simulink model "ZigzagRobot"  (R2025b)
settings: Solver=VariableStepAuto  StartTime=0.0  StopTime=10.0  RelTol=1e-3
values from neighbouring files (symbols this model uses):
  grid_resolution = 100    [ZigZag_robot_simulation.m]
  initial_radius = R0    (= 1)    [ZigZag_robot_simulation.m]
  Kd_w = 0    [ZigZag_robot_simulation.m]
  Ki_w = 50    [ZigZag_robot_simulation.m]
  Kp_w = 10    [ZigZag_robot_simulation.m]
  L_ax = 0.2    [ZigZag_robot_simulation.m]
  linear_speed_cmd = v_ref_const    (= 0.2)    [ZigZag_robot_simulation.m]
  obs_center = [3; 3]    [ZigZag_robot_simulation.m]
  obstacle_radius = 0.25    [ZigZag_robot_simulation.m]
  r_clean = 0.4    [ZigZag_robot_simulation.m]
  R_w = 0.05    [ZigZag_robot_simulation.m]
  rate_gain = k_R    (= 0.05)    [ZigZag_robot_simulation.m]
  room_length = 20    [ZigZag_robot_simulation.m]
  theta0 = (rand()*2*pi) - pi    [ZigZag_robot_simulation.m]
  x0 = (rand()*room_length) - halfL    [ZigZag_robot_simulation.m]
  y0 = (rand()*room_length) - halfL    [ZigZag_robot_simulation.m]
libraries: slpidlib x2
settings Model: Creator=shubh  LastModifiedBy=shubh

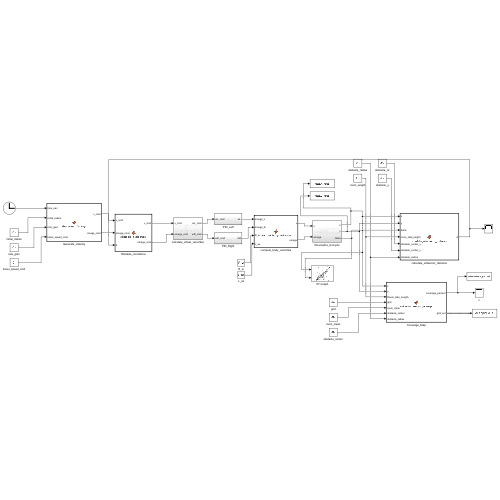
[thumbnail: Simulink's stored preview of the top-level diagram]
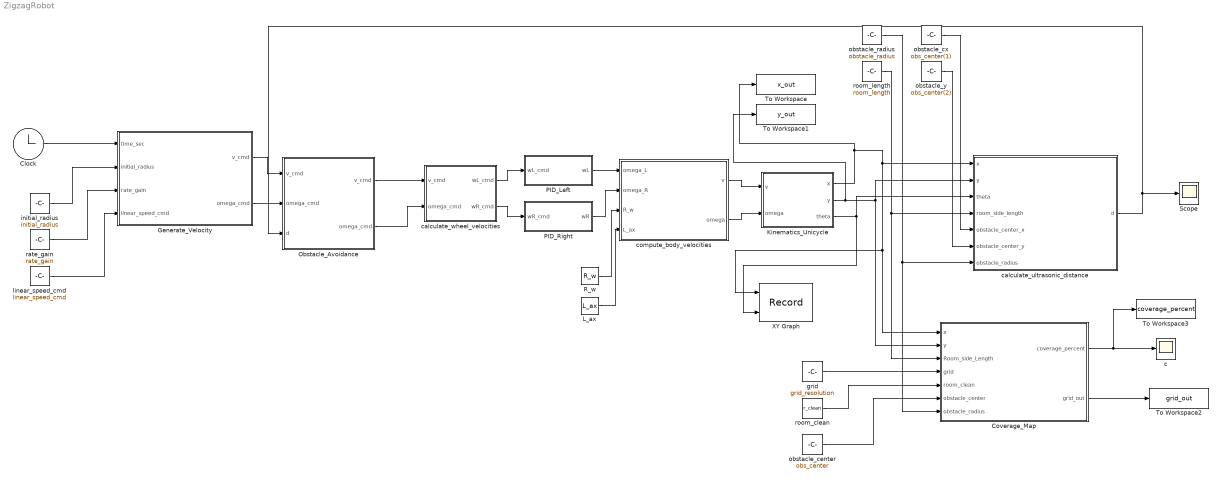
== system ZigzagRobot ==
  Clock : Clock
  Coverage_Map : MATLAB Function  TreatAsAtomicUnit=on
  Generate_Velocity : MATLAB Function  TreatAsAtomicUnit=on
  Kinematics_Unicycle : Subsystem
  L_ax : Constant  Value=L_ax
  Obstacle_Avoidance : MATLAB Function  TreatAsAtomicUnit=on
  PID_Left : Subsystem
  PID_Right : Subsystem
  R_w : Constant  Value=R_w
  Scope : Scope
      settings: ActiveDisplayYMinimum=-1  ActiveDisplayYMaximum=1
  To Workspace : ToWorkspace  VariableName=x_out  SampleTime=-1
  To Workspace1 : ToWorkspace  VariableName=y_out  SampleTime=-1
  To Workspace2 : ToWorkspace  VariableName=grid_out  SaveFormat=Timeseries  SampleTime=-1
  To Workspace3 : ToWorkspace  VariableName=coverage_percent  SaveFormat=Timeseries  SampleTime=-1
  XY Graph : Record  NumPorts=2.0  FileSettingsInternal="{\"entries\":[{\"content\":{\"excelSettings\":{\"content\":{},\"type\":\"Streamout.ExcelSettings\"},\"parquetSettings\":{\"content\":{},\"type\":\"Streamout.ParquetSettings\"}},\"type\":\"Streamout.FileSettingStorage\",\"uuid\":\"\"}],\"packageUris\":[\"http:\\/\\/schema.mathworks.com\\/mf0\\/streamout_blocks\\/R2020a\"],\"version\":\"1.0\"}"  FrameSettings=[0, 0]  Layout=[1 1]  SignalsInternal="{\"entries\":[{\"content\":{\"signals\":[{\"content\":{\"blockPath\":[],\"dimensions\":[1],\"domain\":\"\",\"lineColor\":\"#a2142f\",\"plots\":[ 1 ],\"port\":1,\"signalID\":1,\"signalName\":\"Kinematics_Unicycle:1\"},\"type\":\"RecordBlkView.Signal\",\"uuid\":\"\"},{\"content\":{\"blockPath\":[],\"dimensions\":[1],\"domain\":\"\",\"lineColor\":\"#139fff\",\"plots\":[ 1 ],\"port\":2,\"signalID\":2,\"signalName\":\"Kinematics_Unicycle:3\"},\"type\":\"RecordBlkView.Signal\",\"uuid\":\"\"}]},\"type\":\"RecordBlkView.InputSignals\",\"uuid\":\"\"}],\"packageUris\":[\"http:\\/\\/schema.mathworks.com\\/mf0\\/streamout_blocks\\/R2020a\"],\"version\":\"1.0\"}"  VisualizationBindings="{\"xyplotplugin\":{\"info\":[{\"series\":[{\"bindingParametersList\":[{\"parameter\":\"X-Axis\",\"signalID\":1,\"signalName\":\"Kinematics_Unicycle:1\"},{\"parameter\":\"Y-Axis\",\"signalID\":2,\"signalName\":\"Kinematics_Unicycle:3\"}],\"seriesID\":0}],\"subplotID\":1}]}}"  CompatibilityTag=XY
  c : Scope
      settings: ActiveDisplayYMinimum=-1  ActiveDisplayYMaximum=1
  calculate_ultrasonic_distance : MATLAB Function  TreatAsAtomicUnit=on
  calculate_wheel_velocities : Subsystem
  compute_body_velocities : MATLAB Function  TreatAsAtomicUnit=on
  grid : Constant  Value=grid_resolution
  initial_radius : Constant  Value=initial_radius
  linear_speed_cmd : Constant  Value=linear_speed_cmd
  obstacle_center : Constant  Value=obs_center
  obstacle_cx : Constant  Value=obs_center(1)
  obstacle_radius : Constant  Value=obstacle_radius
  obstacle_y : Constant  Value=obs_center(2)
  rate_gain : Constant  Value=rate_gain
  room_clean : Constant  Value=r_clean
  room_length : Constant  Value=room_length
  wires:
  linear_speed_cmd/1 -> Generate_Velocity/4(linear_speed_cmd)
  calculate_wheel_velocities/1(wL_cmd) -> PID_Left/1(wL_cmd)
  Coverage_Map/2(grid_out) -> To Workspace2/1
  Obstacle_Avoidance/1(v_cmd) -> calculate_wheel_velocities/1(v_cmd)
  room_clean/1 -> Coverage_Map/5(room_clean)
  PID_Right/1(wR) -> compute_body_velocities/2(omega_R)
  Kinematics_Unicycle/2(y) -> To Workspace1/1, calculate_ultrasonic_distance/2(y), Coverage_Map/2(y)
  calculate_ultrasonic_distance/1(d) -> Obstacle_Avoidance/3(d), Scope/1
  room_length/1 -> Coverage_Map/3(Room_side_Length), calculate_ultrasonic_distance/4(room_side_length)
  Obstacle_Avoidance/2(omega_cmd) -> calculate_wheel_velocities/2(omega_cmd)
  L_ax/1 -> compute_body_velocities/4(L_ax)
  obstacle_y/1 -> calculate_ultrasonic_distance/6(obstacle_center_y)
  obstacle_center/1 -> Coverage_Map/6(obstacle_center)
  grid/1 -> Coverage_Map/4(grid)
  Generate_Velocity/1(v_cmd) -> Obstacle_Avoidance/1("v_cmd ")
  obstacle_cx/1 -> calculate_ultrasonic_distance/5(obstacle_center_x)
  calculate_wheel_velocities/2(wR_cmd) -> PID_Right/1(wR_cmd)
  rate_gain/1 -> Generate_Velocity/3(rate_gain)
  Clock/1 -> Generate_Velocity/1(time_sec)
  Kinematics_Unicycle/1(x) -> Coverage_Map/1(x), XY Graph/1, calculate_ultrasonic_distance/1(x), To Workspace/1
  Kinematics_Unicycle/3(theta) -> calculate_ultrasonic_distance/3(theta), XY Graph/2
  PID_Left/1(wL) -> compute_body_velocities/1(omega_L)
  obstacle_radius/1 -> calculate_ultrasonic_distance/7(obstacle_radius), Coverage_Map/7(obstacle_radius)
  Generate_Velocity/2(omega_cmd) -> Obstacle_Avoidance/2("omega_cmd ")
  Coverage_Map/1(coverage_percent) -> To Workspace3/1, c/1
  R_w/1 -> compute_body_velocities/3(R_w)
  compute_body_velocities/2(omega) -> Kinematics_Unicycle/2(omega)
  compute_body_velocities/1(v) -> Kinematics_Unicycle/1(v)
  initial_radius/1 -> Generate_Velocity/2(initial_radius)

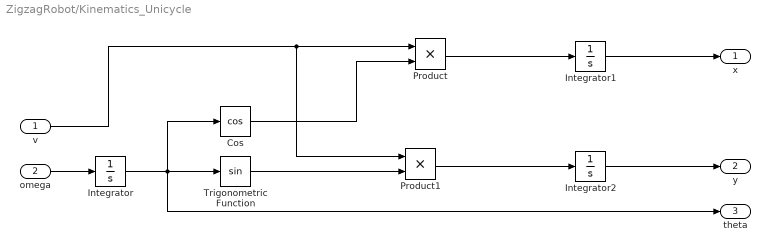
== system ZigzagRobot/Kinematics_Unicycle ==
  v : Inport
  omega : Inport  Port=2
  Cos : Trigonometry  Operator=cos
  Integrator : Integrator  InitialCondition=theta0
  Integrator1 : Integrator  InitialCondition=x0
  Integrator2 : Integrator  InitialCondition=y0
  Product : Product
  Product1 : Product
  Trigonometric Function : Trigonometry
  x : Outport
  y : Outport  Port=2  VectorParamsAs1DForOutWhenUnconnected=off
  theta : Outport  Port=3  VectorParamsAs1DForOutWhenUnconnected=off
  wires:
  omega/1 -> Integrator/1
  Integrator/1 -> theta/1, Trigonometric Function/1, Cos/1
  v/1 -> Product1/1, Product/1
  Cos/1 -> Product/2
  Trigonometric Function/1 -> Product1/2
  Product/1 -> Integrator1/1
  Product1/1 -> Integrator2/1
  Integrator1/1 -> x/1
  Integrator2/1 -> y/1

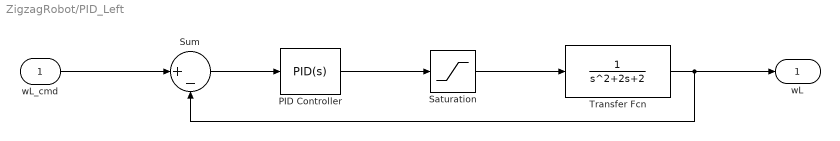
== system ZigzagRobot/PID_Left ==
  wL_cmd : Inport
  PID Controller : slpidlib/PID Controller  Controller=PID  Form=Parallel  TimeDomain=Continuous-time  UseExternalTs=off  SampleTime=-1  IntegratorMethod=Forward Euler  FilterMethod=Forward Euler  ControllerParametersSource=internal  P=Kp_w  I=Ki_w  UseKiTs=off  D=Kd_w  UseExternalDerivativeSource=off  N=100  UseFilter=on  TunerSelectOption=Transfer Function Based (PID Tuner App)  InitialConditionSource=internal  InitialConditionForIntegrator=0  InitialConditionForFilter=0  DifferentiatorICPrevScaledInput=0  ExternalReset=none  TrackingMode=off  Kt=1  LimitOutput=off  SatLimitsSource=internal  UpperSaturationLimit=inf  LowerSaturationLimit=-inf  LinearizeAsGain=on  AntiWindupMode=none  Kb=1  LimitIntegrator=off  UpperIntegratorSaturationLimit=inf  LowerIntegratorSaturationLimit=-inf  POutMin=[]  POutMax=[]  IOutMin=[]  IOutMax=[]  DOutMin=[]  DOutMax=[]  NOutMin=[]  NOutMax=[]  SumOutMin=[]  SumOutMax=[]  SaturationOutMin=[]  SaturationOutMax=[]  PParamMin=[]  PParamMax=[]  IParamMin=[]  IParamMax=[]  DParamMin=[]  DParamMax=[]  NParamMin=[]  NParamMax=[]  KbParamMin=[]  KbParamMax=[]  KtParamMin=[]  KtParamMax=[]  KbOutMin=[]  KbOutMax=[]  KtOutMin=[]  KtOutMax=[]  IntegratorOutMin=[]  IntegratorOutMax=[]  FilterOutMin=[]  FilterOutMax=[]  SumI1OutMin=[]  SumI1OutMax=[]  SumI2OutMin=[]  SumI2OutMax=[]  SumI3OutMin=[]  SumI3OutMax=[]  SumI4OutMin=[]  SumI4OutMax=[]  SumDOutMin=[]  SumDOutMax=[]  DifferentiatorOutMin=[]  DifferentiatorOutMax=[]  FilterDiffOutCoefMin=[]  FilterDiffOutCoefMax=[]  ReciprocalOutMin=[]  ReciprocalOutMax=[]  SumDenOutMin=[]  SumDenOutMax=[]  SumNumOutMin=[]  SumNumOutMax=[]  DivideOutMin=[]  DivideOutMax=[]  UdiffTsProdOutMin=[]  UdiffTsProdOutMax=[]  NTsProdOutMin=[]  NTsProdOutMax=[]  UintegralTsProdOutMin=[]  UintegralTsProdOutMax=[]  UngainTsProdOutMin=[]  UngainTsProdOutMax=[]  ClampingZeroOutDataTypeStr=Inherit: Inherit via back propagation  ClampingZeroOutMin=[]  ClampingZeroOutMax=[]  FilterDenConstantOutDataTypeStr=Inherit: Inherit via back propagation  FilterDenConstantOutMin=[]  FilterDenConstantOutMax=[]  PCopyOutDataTypeStr=Inherit: Inherit via back propagation  PCopyOutMin=[]  PCopyOutMax=[]  NCopyOutDataTypeStr=Inherit: Inherit via back propagation  NCopyOutMin=[]  NCopyOutMax=[]  IntegratorContinuousStateAttributes=''  IntegratorStateMustResolveToSignalObject=off  IntegratorRTWStateStorageClass=Auto  FilterContinuousStateAttributes=''  FilterStateMustResolveToSignalObject=off  FilterRTWStateStorageClass=Auto  ParallelPVariant=InternalParameters  IdealPVariant=Disabled  IVariant=InternalParameters  DVariant=InternalParameters  IntegratorVariant=Continuous  SatVariant=Disabled  AWVariant=Passthrough  PCopyVariant=Disabled  TRVariant=Disabled  FdbkBlocksVariant=Forward  IdealPFdbkVariant=Disabled  SatFdbkVariant=Disabled  DerivativeFilterVariant=ContFilter  NVariant=InternalParameters  NCopyVariant=Disabled  FilterICVariant=InternalICsFilter  IntegratorICVariant=InternalICs  ExternalResetVariant=Disabled  TRSumVariant=Passthrough  SumFdbkVariant=Disabled  SumVariant=Sum_PID  TsampFilterVariant=InternalTs  TsampNgainVariant=Passthrough  TsampIntegralVariant=Disabled_SignalSpec  ExternalSaturationOutDataTypeStr=Inherit: Same as second input  DerivativeSourceVariant=ErrorSignal  PreIntVariant=InternalPreInt
  Saturation : Saturate  UpperLimit=12  LowerLimit=-12
  Sum : Sum  Inputs=|+-
  Transfer Fcn : TransferFcn  Denominator=[1 2 2]
  wL : Outport
  wires:
  Transfer Fcn/1 -> Sum/2, wL/1
  wL_cmd/1 -> Sum/1
  Sum/1 -> PID Controller/1
  PID Controller/1 -> Saturation/1
  Saturation/1 -> Transfer Fcn/1

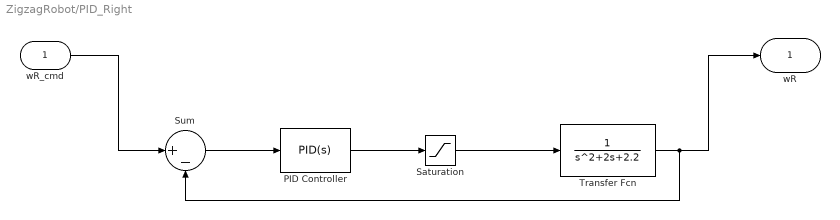
== system ZigzagRobot/PID_Right ==
  wR_cmd : Inport
  PID Controller : slpidlib/PID Controller  Controller=PID  Form=Parallel  TimeDomain=Continuous-time  UseExternalTs=off  SampleTime=-1  IntegratorMethod=Forward Euler  FilterMethod=Forward Euler  ControllerParametersSource=internal  P=Kp_w  I=Ki_w  UseKiTs=off  D=Kd_w  UseExternalDerivativeSource=off  N=100  UseFilter=on  TunerSelectOption=Transfer Function Based (PID Tuner App)  InitialConditionSource=internal  InitialConditionForIntegrator=0  InitialConditionForFilter=0  DifferentiatorICPrevScaledInput=0  ExternalReset=none  TrackingMode=off  Kt=1  LimitOutput=off  SatLimitsSource=internal  UpperSaturationLimit=inf  LowerSaturationLimit=-inf  LinearizeAsGain=on  AntiWindupMode=none  Kb=1  LimitIntegrator=off  UpperIntegratorSaturationLimit=inf  LowerIntegratorSaturationLimit=-inf  POutMin=[]  POutMax=[]  IOutMin=[]  IOutMax=[]  DOutMin=[]  DOutMax=[]  NOutMin=[]  NOutMax=[]  SumOutMin=[]  SumOutMax=[]  SaturationOutMin=[]  SaturationOutMax=[]  PParamMin=[]  PParamMax=[]  IParamMin=[]  IParamMax=[]  DParamMin=[]  DParamMax=[]  NParamMin=[]  NParamMax=[]  KbParamMin=[]  KbParamMax=[]  KtParamMin=[]  KtParamMax=[]  KbOutMin=[]  KbOutMax=[]  KtOutMin=[]  KtOutMax=[]  IntegratorOutMin=[]  IntegratorOutMax=[]  FilterOutMin=[]  FilterOutMax=[]  SumI1OutMin=[]  SumI1OutMax=[]  SumI2OutMin=[]  SumI2OutMax=[]  SumI3OutMin=[]  SumI3OutMax=[]  SumI4OutMin=[]  SumI4OutMax=[]  SumDOutMin=[]  SumDOutMax=[]  DifferentiatorOutMin=[]  DifferentiatorOutMax=[]  FilterDiffOutCoefMin=[]  FilterDiffOutCoefMax=[]  ReciprocalOutMin=[]  ReciprocalOutMax=[]  SumDenOutMin=[]  SumDenOutMax=[]  SumNumOutMin=[]  SumNumOutMax=[]  DivideOutMin=[]  DivideOutMax=[]  UdiffTsProdOutMin=[]  UdiffTsProdOutMax=[]  NTsProdOutMin=[]  NTsProdOutMax=[]  UintegralTsProdOutMin=[]  UintegralTsProdOutMax=[]  UngainTsProdOutMin=[]  UngainTsProdOutMax=[]  ClampingZeroOutDataTypeStr=Inherit: Inherit via back propagation  ClampingZeroOutMin=[]  ClampingZeroOutMax=[]  FilterDenConstantOutDataTypeStr=Inherit: Inherit via back propagation  FilterDenConstantOutMin=[]  FilterDenConstantOutMax=[]  PCopyOutDataTypeStr=Inherit: Inherit via back propagation  PCopyOutMin=[]  PCopyOutMax=[]  NCopyOutDataTypeStr=Inherit: Inherit via back propagation  NCopyOutMin=[]  NCopyOutMax=[]  IntegratorContinuousStateAttributes=''  IntegratorStateMustResolveToSignalObject=off  IntegratorRTWStateStorageClass=Auto  FilterContinuousStateAttributes=''  FilterStateMustResolveToSignalObject=off  FilterRTWStateStorageClass=Auto  ParallelPVariant=InternalParameters  IdealPVariant=Disabled  IVariant=InternalParameters  DVariant=InternalParameters  IntegratorVariant=Continuous  SatVariant=Disabled  AWVariant=Passthrough  PCopyVariant=Disabled  TRVariant=Disabled  FdbkBlocksVariant=Forward  IdealPFdbkVariant=Disabled  SatFdbkVariant=Disabled  DerivativeFilterVariant=ContFilter  NVariant=InternalParameters  NCopyVariant=Disabled  FilterICVariant=InternalICsFilter  IntegratorICVariant=InternalICs  ExternalResetVariant=Disabled  TRSumVariant=Passthrough  SumFdbkVariant=Disabled  SumVariant=Sum_PID  TsampFilterVariant=InternalTs  TsampNgainVariant=Passthrough  TsampIntegralVariant=Disabled_SignalSpec  ExternalSaturationOutDataTypeStr=Inherit: Same as second input  DerivativeSourceVariant=ErrorSignal  PreIntVariant=InternalPreInt
  Saturation : Saturate  UpperLimit=12  LowerLimit=-12
  Sum : Sum  Inputs=|+-
  Transfer Fcn : TransferFcn  Denominator=[1 2 2.2]
  wR : Outport
  wires:
  Sum/1 -> PID Controller/1
  PID Controller/1 -> Saturation/1
  Transfer Fcn/1 -> Sum/2, wR/1
  wR_cmd/1 -> Sum/1
  Saturation/1 -> Transfer Fcn/1

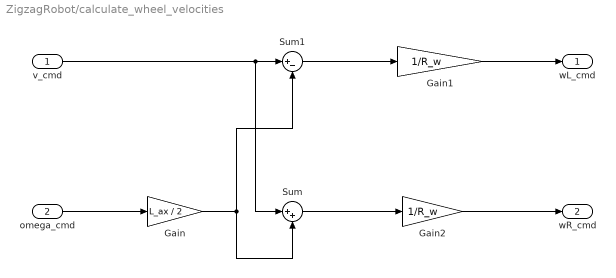
== system ZigzagRobot/calculate_wheel_velocities ==
  v_cmd : Inport
  omega_cmd : Inport  Port=2
  Gain : Gain  Gain=L_ax / 2
  Gain1 : Gain  Gain=1/R_w
  Gain2 : Gain  Gain=1/R_w
  Sum : Sum  Inputs=|++
  Sum1 : Sum  Inputs=|+-
  wL_cmd : Outport
  wR_cmd : Outport  Port=2  VectorParamsAs1DForOutWhenUnconnected=off
  wires:
  omega_cmd/1 -> Gain/1
  v_cmd/1 -> Sum/1, Sum1/1
  Gain/1 -> Sum1/2, Sum/2
  Sum/1 -> Gain2/1
  Sum1/1 -> Gain1/1
  Gain1/1 -> wL_cmd/1
  Gain2/1 -> wR_cmd/1

== matlab function ZigzagRobot/Coverage_Map ==
  settings: updateMethod=DISCRETE  sampleTime=Ts
  data: x input; coverage_percent output; y input; Room_side_Length input; grid input; grid_out output size=[100 100]; room_clean input; obstacle_center input; obstacle_radius input
function [coverage_percent, grid_out] = calculate_coverage_map( ...
            x, y, Room_side_Length, grid, room_clean, obstacle_center, obstacle_radius)
%#codegen
% Calculates and updates the coverage map and computes the percentage of the room cleaned.
%
% Inputs:
% x, y: Current robot position (m)
% Room_side_Length: Side length of the square room (m)
% grid: Resolution of the grid (grid x grid)
% r_clean: Robot's cleaning radius (m)
% obstacle_center: [x, y] center of the obstacle
% obstacle_radius: Radius of the circular obstacle
%
% Outputs:
% coverage_percent: Percentage of cleanable area that has been cleaned (%)
% grid_out: The final updated coverage grid

persistent grid_initialized coverage_grid

if isempty(grid_initialized)
    coverage_grid = zeros(grid, grid);
    halfL = Room_side_Length / 2;
    cell_size = Room_side_Length / grid;
    
    % Mark obstacle cells
    for i = 1:grid
        for j = 1:grid
            center_x = (i-0.5)*cell_size - halfL;
            center_y = (j-0.5)*cell_size - halfL;
            dist_to_obs_center = sqrt((center_x - obstacle_center(1))^2 + (center_y - obstacle_center(2))^2);
            if dist_to_obs_center <= obstacle_radius
                coverage_grid(i,j) = -1;
            end
        end
    end
    grid_initialized = true;
end

halfL = Room_side_Length / 2;
cell_size = Room_side_Length / grid;

if x >= -halfL && x <= halfL && y >= -halfL && y <= halfL
    ic = floor((x + halfL) / cell_size) + 1;
    jc = floor((y + halfL) / cell_size) + 1;
    
    if ic<1 || ic>grid || jc<1 || jc>grid
        grid_out = coverage_grid;
        total_cells = nnz(coverage_grid ~= -1);
        coverage_percent = 100 * nnz(coverage_grid == 1) / total_cells;
        return;
    end
    
    n_cells_radius = ceil(room_clean / cell_size);
    
    for i = ic - n_cells_radius : ic + n_cells_radius
        for j = jc - n_cells_radius : jc + n_cells_radius
            if i >= 1 && i <= grid && j >= 1 && j <= grid
                if coverage_grid(i,j) == -1
                    continue;
                end
                center_x = (i-0.5)*cell_size - halfL;
                center_y = (j-0.5)*cell_size - halfL;
                if sqrt((center_x - x)^2 + (center_y - y)^2) <= room_clean
                    coverage_grid(i,j) = 1;
                end
            end
        end
    end
end

grid_out = coverage_grid;
total_cleanable_cells = nnz(coverage_grid ~= -1);
if total_cleanable_cells > 0
    coverage_percent = 100 * nnz(coverage_grid == 1) / total_cleanable_cells;
else
    coverage_percent = 0;
end

end

== matlab function ZigzagRobot/calculate_ultrasonic_distance ==
  data: x input; d output; y input; theta input; room_side_length input; obstacle_center_x input; obstacle_center_y input; obstacle_radius input
function d = calculate_ultrasonic_distance( ...
            x, y, theta, room_side_length, obstacle_center_x, obstacle_center_y, obstacle_radius)
%#codegen
% Calculates the distance (d) to the nearest obstacle (wall or cylinder) 
% along the robot's heading (theta).
% The square room extends from -room_side_length/2 to +room_side_length/2.

room_half_size = room_side_length/2;

% Direction vector of the measurement ray (along the robot's x-axis)
ray_dir_x = cos(theta);
ray_dir_y = sin(theta);

% Initialize minimum distance to a very large value
min_distance = 1e6;

%% --- Intersection with Walls (Ray-Line Segment Intersection) ---
% A point on the ray is P(t) = (x, y) + t * (ray_dir_x, ray_dir_y)
% t represents the distance from the robot to the intersection point.

% 1. Wall x = +room_half_size (Right Wall)
if abs(ray_dir_x) > 1e-6 % Check if ray is not parallel to the wall
    t_param = (room_half_size - x) / ray_dir_x;
    if t_param > 0 % Intersection is in front of the robot
        intersection_y = y + t_param * ray_dir_y;
        if abs(intersection_y) <= room_half_size % Intersection is within the wall bounds
            min_distance = min(min_distance, t_param);
        end
    end
end

% 2. Wall x = -room_half_size (Left Wall)
if abs(ray_dir_x) > 1e-6
    t_param = (-room_half_size - x) / ray_dir_x;
    if t_param > 0
        intersection_y = y + t_param * ray_dir_y;
        if abs(intersection_y) <= room_half_size
            min_distance = min(min_distance, t_param);
        end
    end
end

% 3. Wall y = +room_half_size (Top Wall)
if abs(ray_dir_y) > 1e-6
    t_param = (room_half_size - y) / ray_dir_y;
    if t_param > 0
        intersection_x = x + t_param * ray_dir_x;
        if abs(intersection_x) <= room_half_size
            min_distance = min(min_distance, t_param);
        end
    end
end

% 4. Wall y = -room_half_size (Bottom Wall)
if abs(ray_dir_y) > 1e-6
    t_param = (-room_half_size - y) / ray_dir_y;
    if t_param > 0
        intersection_x = x + t_param * ray_dir_x;
        if abs(intersection_x) <= room_half_size
            min_distance = min(min_distance, t_param);
        end
    end
end

%% --- Intersection with the Cylinder (Ray-Sphere Intersection) ---
center_x = obstacle_center_x;
center_y = obstacle_center_y;

% Define quadratic equation terms A*t^2 + B*t + C = 0 for intersection
A_coeff = ray_dir_x^2 + ray_dir_y^2;

vector_x = x - center_x;
vector_y = y - center_y;

B_coeff = 2 * (ray_dir_x * vector_x + ray_dir_y * vector_y);

C_coeff = vector_x^2 + vector_y^2 - obstacle_radius^2;

% Calculate the discriminant
discriminant = B_coeff^2 - 4 * A_coeff * C_coeff;

if discriminant >= 0 % If discriminant is non-negative, there is an intersection
    sqrt_disc = sqrt(discriminant);
    
    t1 = (-B_coeff + sqrt_disc) / (2 * A_coeff);
    t2 = (-B_coeff - sqrt_disc) / (2 * A_coeff);
    
    % Only consider intersections in front of the robot (t > 0)
    if t1 > 0
        min_distance = min(min_distance, t1);
    end
    if t2 > 0
        min_distance = min(min_distance, t2);
    end
end

%% Final Result
if min_distance == 1e6
    d = room_side_length;  % No intersection found, return the room side length as a maximum distance
else
    d = min_distance;
end
end

== matlab function ZigzagRobot/Obstacle_Avoidance ==
  settings: updateMethod=DISCRETE
  data: v_cmd input; v_cmd output; omega_cmd input; d input; omega_cmd output
function [v_cmd, omega_cmd] = obstacle_avoidance(v_cmd, omega_cmd, d)
%#codegen
% Decides between the spiral trajectory and an avoidance maneuver.

% Define thresholds (Constants, adjust as needed)
d_warn = 1.0; % Warning zone: approach the wall/obstacle (start of avoidance maneuver)
d_stop = 0.4; % Critical zone: must turn immediately

% Avoidance parameters
omega_turn_soft = 0.6; % Gentle turn rate (rad/s)
omega_turn_hard = 1.5; % Sharp turn rate (rad/s)
v_turn_reduction = 0.6; % Speed reduction factor (applied in critical zone)

% Persistent state for avoidance direction: 
% 1 = Left, -1 = Right, 0 = Reset/Needs new choice (Fixed size scalar)
persistent turn_direction;

% Initialize persistent variable if it's empty (first run)
if isempty(turn_direction)
    turn_direction = 0; % Initialize to reset state (0)
end

% 1. Normal Case: Far from obstacle (d > d_warn)
if d > d_warn
    % Reset turn direction (set to 0) for the next avoidance maneuver
    turn_direction = 0;
    
    return;
end

% Check if a new turn direction needs to be chosen (only happens when turn_direction is 0)
if turn_direction == 0
    % Randomly commit to a turn direction (Left: 1 or Right: -1)
    if rand() > 0.5
        turn_direction = 1; 
    else
        turn_direction = -1;
    end
end

% 2. Critical Zone: Must turn sharply (d <= d_stop)
if d <= d_stop
    % Slow down significantly and apply a hard turn based on the committed direction
    v_cmd = v_cmd * v_turn_reduction; 
    omega_cmd = turn_direction * omega_turn_hard;
    return;
end

% 3. Warning Zone: Approach detected (d_stop < d <= d_warn)
% The robot maintains the committed turn direction (turn_direction is non-zero here)
if d > d_stop && d <= d_warn
    % Slow down slightly and apply a soft turn in the committed direction
    v_cmd = v_cmd * 0.8; % Slight speed reduction
    omega_cmd = turn_direction * omega_turn_soft;
    return;
end

% Fallback 
end

== matlab function ZigzagRobot/Generate_Velocity ==
  data: time_sec input; v_cmd output; initial_radius input; rate_gain input; linear_speed_cmd input; omega_cmd output
function [v_cmd, omega_cmd] = Generate_Velocity(time_sec, initial_radius, rate_gain, linear_speed_cmd)
%#codegen
% This function implements a Spiral Trajectory Law.
% R = R0 + k_R * t
% omega = v / R

% 1. Calculate the current radius of curvature (R)
current_radius = initial_radius + rate_gain * time_sec;

% 2. Linear Velocity Command (v_cmd)
% The linear velocity is constant
v_cmd = linear_speed_cmd;

% 3. Angular Velocity Command (omega_cmd)
% omega = v / R
omega_cmd = linear_speed_cmd / current_radius;

end

== matlab function ZigzagRobot/compute_body_velocities ==
  data: omega_L input; v output; omega_R input; R_w input; L_ax input; omega output
function [v, omega] = compute_body_velocities(omega_L, omega_R, R_w, L_ax)
%#codegen
% Computes the robot's linear velocity (v) and angular velocity (omega)
% from the angular velocities of the left and right wheels (omega_L, omega_R).
%
% This implements the unicycle inverse kinematic model:
% v     = (R_w / 2) * (omega_R + omega_L)
% omega = (R_w / L_ax) * (omega_R - omega_L)
%
% Inputs:
% omega_L: Angular velocity of the Left wheel (rad/s)
% omega_R: Angular velocity of the Right wheel (rad/s)
% R_w: Wheel radius (m)
% L_ax: Axle track (distance between wheels) (m)
%
% Outputs:
% v: Robot's linear velocity (m/s)
% omega: Robot's angular velocity (rad/s)

% 1. Calculate Linear Velocity (v)
v = (R_w / 2) * (omega_R + omega_L);

% 2. Calculate Angular Velocity (omega)
omega = (R_w / L_ax) * (omega_R - omega_L);

end
